simulink model "G474_Mode2_Direct_Start_Repair"  (R2024b)
settings: Solver=FixedStepDiscrete  StartTime=0.0  StopTime=q.stop_time  FixedStep=p.Ts  RelTol=1e-3
InitFcn:
  | m2_project_root=fileparts(fileparts(get_param(bdroot,'FileName')));Simulink.fileGenControl('set','CacheFolder',fullfile(m2_project_root,'work'),'CodeGenFolder',fullfile(m2_project_root,'work'),'createDir',true);m2_ws=get_param(bdroot,'ModelWorkspace');m2_q=getVariable(m2_ws,'q');if isfield(m2_q,'random_initial_angle') && m2_q.random_initial_angle,m2_q.initial_theta_e=2*pi*rand();end;m2_q.initial_state=[0;0;m2_q.initial_rpm*2*pi/60;m2_q.initial_theta_e];assignin(m2_ws,'q',m2_q);fprintf('MODE2 physical initial electrical angle: %.9f deg (random=%d)\n',m2_q.initial_theta_e*180/pi,m2_q.random_initial_angle);
model workspace (MAT data in the model file):
  fSin = [0 0.00153398001567 0.00306795700453 0.00460192607716 0.00613588513806 0.00766982883215 0.00920375529677 0.0107376594096 0.0122715383768 0.0138053894043 0.0153392059729 0.0168729871511 ... (1025 elements, 1025x1)]
  p.Rs = 0.875
  p.Ls = 0.0002
  p.Ld = 0.0002
  p.Lq = 0.0002
  p.Flux = 0.00752
  p.MOTOR_POLES = 14
  p.Ts = 5e-05
  p.Gain = 5000
  p.PLL_BW_Hz = 15
  p.Comp_BW_Hz = 5
  p.PLL_kp = 188.495559215
  p.PLL_ki = 0.444132198049
  p.Comp_Kp = 62.8318530718
  p.Comp_Ki = 0.0493480220054
  p.Comp_Mode = 0
  p.SMO_Kslide = 10
  p.SMO_Boundary = 0.002
  p.V_deadtime = 0.3
  p.current_deadband = 0.01
  p.pll_step_limit = 0.157079632679
  p.speed_decimation = 8
  p.speed_filter_old = 0.95
  p.speed_filter_new = 0.05
  q.Ts = 5e-05
  q.Rs = 0.875
  q.Ld = 0.0002
  q.Lq = 0.0002
  q.Flux = 0.00752
  q.pole_pairs = 7
  q.target_rpm = 200
  q.second_rpm = 400
  q.third_rpm = 1000
  q.switch_1 = 0.8
  q.switch_2 = 1.6
  q.Vbus = 12
  q.stop_time = 4
  q.J = 2e-05
  q.B = 1e-05
  q.load_torque = 0.005
  q.load_speed_scale_rad_s = 1
  q.random_initial_angle = 1
  q.initial_theta_e = 0.523598775598
  q.initial_rpm = 0
  q.actual_deadtime_V = 0.3
  q.observer_deadtime_V = 0.3
  q.speed_iq_sign = 1
  q.deadtime_feedforward_V = 0.3
  q.feedforward_start_s = 0.5
  q.feedforward_ramp_s = 0.5
  q.speed_kp = 0.01
  q.speed_ki = 0.0001
  q.current_kp = 0.01
  q.current_ki = 1e-05
  q.iq_limit = 12
  q.reference_filter_hz = 2
  q.reference_start_delay_s = 0.15
  q.ramp_step = 0.05
  q.current_channel_sign = 1
  q.initial_state = [0; 0; 0; 0.523598775598]
  s0.psi_s = [0; 0]
  s0.theta = 0
(part 1 of 2)
settings Model: Creator=QXZ-030079  LastModifiedBy=QXZ-030079
settings DataIOCC: SignalLogging=off

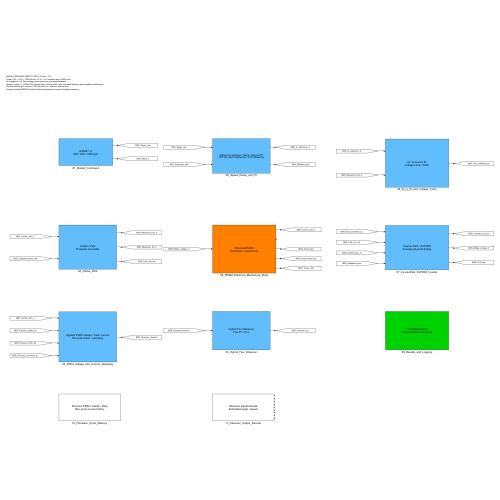
[thumbnail: Simulink's stored preview of the top-level diagram]
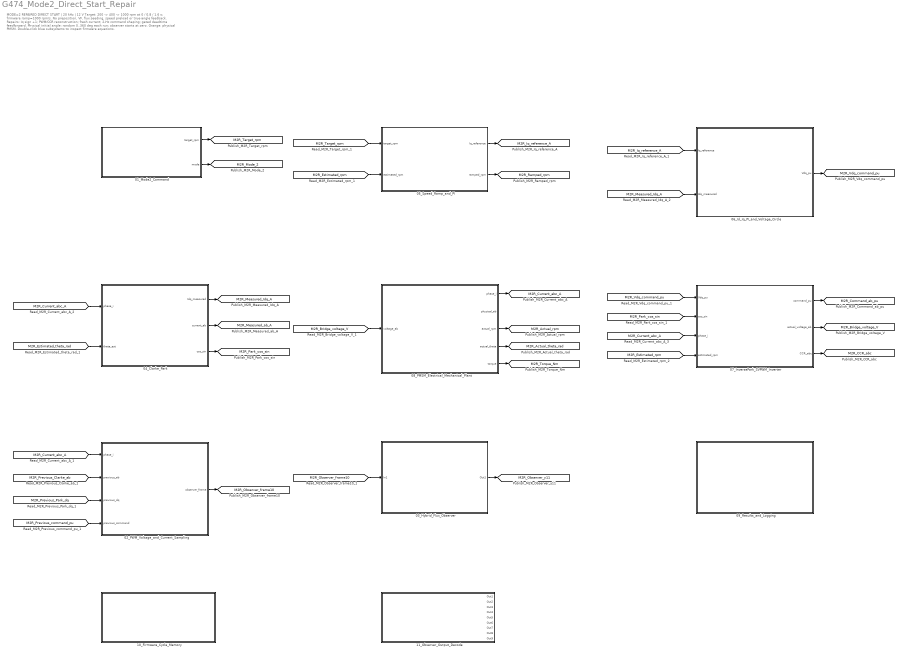
== system G474_Mode2_Direct_Start_Repair ==
  note: MODE=2 REPAIRED DIRECT START | 20 kHz | 12 V
      | Target: 200 -> 400 -> 1000 rpm at 0 / 0.8 / 1.6 s; firmware ramp=1000 rpm/s.
      | No preposition, VF, flux seeding, speed preload or true-angle feedback.
      | Repairs: Iq sign +1; PWM/CCR reconstruction; fresh current; 2-Hz command shaping; gated deadtime feedforward.
      | Physical initial angle: random 0..360 deg each run; observer starts at zero.
      | Orange: physical PMSM. Double-click blue subsystems to inspect firmware equations.
  01_Mode2_Command : Subsystem
      mask Display: disp('MODE = 2\n200 / 400 / 1000 rpm');
  02_PWM_Voltage_and_Current_Sampling : Subsystem
      mask Display: disp('Applied PWM voltage / fresh current\nReconstruction / sampling');
  03_Hybrid_Flux_Observer : Subsystem
      settings: OpenFcn=open_system(gcb,'force')
      mask Display: disp('Hybrid Flux Observer\nFlux PI + PLL');
  04_Clarke_Park : Subsystem
      mask Display: disp('Clarke / Park\nFirmware sine table');
  05_Speed_Ramp_and_PI : Subsystem
      mask Display: disp('Observer warmup / ramp / source PI\n150 ms zero reference / 2 Hz shaping');
  06_Id_Iq_PI_and_Voltage_Circle : Subsystem
      mask Display: disp('Id / Iq source PI\nVoltage circle / OutF');
  07_InversePark_SVPWM_Inverter : Subsystem
      mask Display: disp('Inverse Park / SVPWM\nAverage physical bridge');
  08_PMSM_Electrical_Mechanical_Plant : Subsystem
      mask Display: disp('Physical PMSM\nElectrical + mechanical');
  09_Results_and_Logging : Subsystem
      mask Display: disp('11 labelled scopes\nActual / estimated results');
  10_Firmware_Cycle_Memory : Subsystem
      mask Display: disp('Previous PWM / Clarke / Park\nOne-cycle source history');
  11_Observer_Output_Decode : Subsystem
      mask Display: disp('Observer signal decode\nEstimated angle / speed');
  tag scope: M2R_Actual_rpm=global, M2R_Actual_theta_rad=global, M2R_Bridge_voltage_V=global, M2R_CCR_abc=global, M2R_Command_ab_pu=global, M2R_Current_abc_A=global, M2R_Iq_reference_A=global, M2R_Measured_Idq_A=global, M2R_Measured_ab_A=global, M2R_Mode_2=global, M2R_Observer_frame10=global, M2R_Observer_y11=global, M2R_Park_cos_sin=global, M2R_Ramped_rpm=global, M2R_Target_rpm=global, M2R_Torque_Nm=global, M2R_Vdq_command_pu=global
  wires:
  01_Mode2_Command/2(mode) -> [M2R_Mode_2]
  07_InversePark_SVPWM_Inverter/3(CCR_abc) -> [M2R_CCR_abc]
  05_Speed_Ramp_and_PI/2(ramped_rpm) -> [M2R_Ramped_rpm]
  08_PMSM_Electrical_Mechanical_Plant/5(torque) -> [M2R_Torque_Nm]
  08_PMSM_Electrical_Mechanical_Plant/4(actual_theta) -> [M2R_Actual_theta_rad]
  08_PMSM_Electrical_Mechanical_Plant/3(actual_rpm) -> [M2R_Actual_rpm]
  07_InversePark_SVPWM_Inverter/2(actual_voltage_ab) -> [M2R_Bridge_voltage_V]
  [M2R_Bridge_voltage_V] -> 08_PMSM_Electrical_Mechanical_Plant/1(voltage_ab)
  04_Clarke_Park/3(cos_sin) -> [M2R_Park_cos_sin]
  [M2R_Park_cos_sin] -> 07_InversePark_SVPWM_Inverter/2(cos_sin)
  06_Id_Iq_PI_and_Voltage_Circle/1(Vdq_pu) -> [M2R_Vdq_command_pu]
  [M2R_Vdq_command_pu] -> 07_InversePark_SVPWM_Inverter/1(Vdq_pu)
  05_Speed_Ramp_and_PI/1(Iq_reference) -> [M2R_Iq_reference_A]
  [M2R_Iq_reference_A] -> 06_Id_Iq_PI_and_Voltage_Circle/1(Iq_reference)
  [M2R_Estimated_rpm] -> 05_Speed_Ramp_and_PI/2(estimated_rpm)
  [M2R_Estimated_rpm] -> 07_InversePark_SVPWM_Inverter/4(estimated_rpm)
  01_Mode2_Command/1(target_rpm) -> [M2R_Target_rpm]
  [M2R_Target_rpm] -> 05_Speed_Ramp_and_PI/1(target_rpm)
  [M2R_Estimated_theta_rad] -> 04_Clarke_Park/2(theta_est)
  03_Hybrid_Flux_Observer/1(Out1) -> [M2R_Observer_y11]
  02_PWM_Voltage_and_Current_Sampling/1(observer_frame) -> [M2R_Observer_frame10]
  [M2R_Observer_frame10] -> 03_Hybrid_Flux_Observer/1(In1)
  [M2R_Previous_command_pu] -> 02_PWM_Voltage_and_Current_Sampling/4(previous_command)
  [M2R_Previous_Park_dq] -> 02_PWM_Voltage_and_Current_Sampling/3(previous_dq)
  [M2R_Previous_Clarke_ab] -> 02_PWM_Voltage_and_Current_Sampling/2(previous_ab)
  08_PMSM_Electrical_Mechanical_Plant/1(phase_i) -> [M2R_Current_abc_A]
  [M2R_Current_abc_A] -> 02_PWM_Voltage_and_Current_Sampling/1(phase_i)
  [M2R_Current_abc_A] -> 04_Clarke_Park/1(phase_i)
  [M2R_Current_abc_A] -> 07_InversePark_SVPWM_Inverter/3(phase_i)
  04_Clarke_Park/1(Idq_measured) -> [M2R_Measured_Idq_A]
  [M2R_Measured_Idq_A] -> 06_Id_Iq_PI_and_Voltage_Circle/2(Idq_measured)
  04_Clarke_Park/2(current_ab) -> [M2R_Measured_ab_A]
  07_InversePark_SVPWM_Inverter/1(command_pu) -> [M2R_Command_ab_pu]

== system G474_Mode2_Direct_Start_Repair/01_Mode2_Command ==
  Initial_200rpm : Constant  Value=q.target_rpm
  MODE_SENSORLESS_2 : Constant  Value=2
  Speed_schedule : Sum  Inputs=+++
  Switch_to_1000rpm : Step  Time=q.switch_2  After=q.third_rpm-q.second_rpm  SampleTime=p.Ts
  Switch_to_400rpm : Step  Time=q.switch_1  After=q.second_rpm-q.target_rpm  SampleTime=p.Ts
  target_rpm : Outport
  mode : Outport  Port=2
  wires:
  MODE_SENSORLESS_2/1 -> mode/1
  Speed_schedule/1 -> target_rpm/1
  Initial_200rpm/1 -> Speed_schedule/1
  Switch_to_400rpm/1 -> Speed_schedule/2
  Switch_to_1000rpm/1 -> Speed_schedule/3

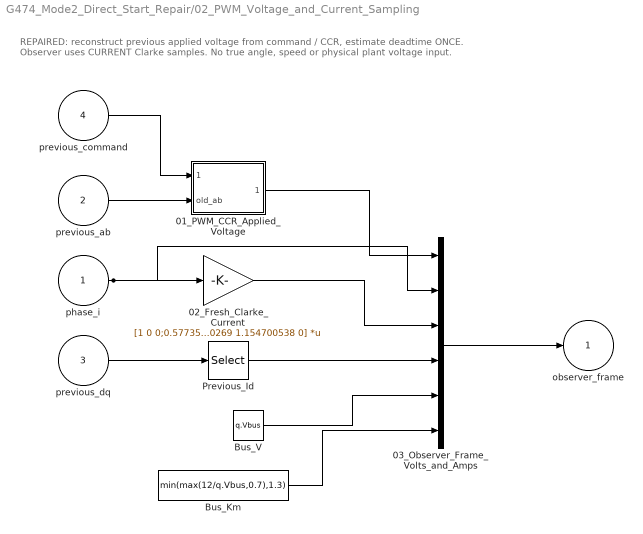
== system G474_Mode2_Direct_Start_Repair/02_PWM_Voltage_and_Current_Sampling ==
  note: REPAIRED: reconstruct previous applied voltage from command / CCR, estimate deadtime ONCE.
      | Observer uses CURRENT Clarke samples. No true angle, speed or physical plant voltage input.
  phase_i : Inport
  previous_ab : Inport  Port=2
  previous_dq : Inport  Port=3
  previous_command : Inport  Port=4
  01_PWM_CCR_Applied_Voltage : MATLAB Function  TreatAsAtomicUnit=on
  02_Fresh_Clarke_Current : Gain  Gain=[1 0 0;0.577350269 1.154700538 0]  Multiplication=Matrix(K*u)
  03_Observer_Frame_Volts_and_Amps : Mux  Inputs=6
  Bus_Km : Constant  Value=min(max(12/q.Vbus,0.7),1.3)
  Bus_V : Constant  Value=q.Vbus
  Previous_Id : Selector  InputPortWidth=2  IndexOptions=Index vector (dialog)  Indices=1  OutputSizes=1
  observer_frame : Outport
  wires:
  01_PWM_CCR_Applied_Voltage/1(voltage) -> 03_Observer_Frame_Volts_and_Amps/1
  previous_command/1 -> 01_PWM_CCR_Applied_Voltage/1(old_command)
  Previous_Id/1 -> 03_Observer_Frame_Volts_and_Amps/4
  Bus_V/1 -> 03_Observer_Frame_Volts_and_Amps/5
  previous_ab/1 -> 01_PWM_CCR_Applied_Voltage/2(old_ab)
  phase_i/1 -> 03_Observer_Frame_Volts_and_Amps/2, 02_Fresh_Clarke_Current/1
  previous_dq/1 -> Previous_Id/1
  02_Fresh_Clarke_Current/1 -> 03_Observer_Frame_Volts_and_Amps/3
  Bus_Km/1 -> 03_Observer_Frame_Volts_and_Amps/6
  03_Observer_Frame_Volts_and_Amps/1 -> observer_frame/1

== system G474_Mode2_Direct_Start_Repair/03_Hybrid_Flux_Observer ==
  In1 : Inport
  01_Voltage_Compensation : Subsystem
      settings: OpenFcn=open_system(gcb,'force')
      mask Display: port_label('input',1,'command_pu');port_label('input',2,'phase_current');port_label('input',3,'Vbus');port_label('input',4,'Km');port_label('output',1,'voltage_V');
  02_Active_Flux_Models : Subsystem
      settings: OpenFcn=open_system(gcb,'force')
      mask Display: port_label('input',1,'theta_previous');port_label('input',2,'current_ab');port_label('input',3,'psi_s_previous');port_label('input',4,'Id');port_label('output',1,'psi_I');port_label('output',2,'psi_V');
  03_Flux_Feedback : Subsystem
      settings: OpenFcn=open_system(gcb,'force')
      mask Display: port_label('input',1,'psi_I');port_label('input',2,'psi_V');port_label('output',1,'Ucomp');
  04_Stator_Integrator : Subsystem
      settings: OpenFcn=open_system(gcb,'force')
      mask Display: port_label('input',1,'voltage_V');port_label('input',2,'current_ab');port_label('input',3,'Ucomp');port_label('output',1,'psi_s_new');port_label('output',2,'psi_s_previous');
  05_PLL_and_Angle : Subsystem
      settings: OpenFcn=open_system(gcb,'force')
      mask Display: port_label('input',1,'psi_V');port_label('output',1,'theta_previous');port_label('output',2,'step_rad');port_label('output',3,'theta_new');port_label('output',4,'PLL_error');
  06_Speed_Filter : Subsystem
      settings: OpenFcn=open_system(gcb,'force')
      mask Display: port_label('input',1,'step_rad');port_label('output',1,'electrical_Hz');port_label('output',2,'firmware_RPM');
  Input split : Demux  Outputs=[2 3 2 1 1 1]
  Results : Mux  Inputs=8
  Out1 : Outport
  wires:
  03_Flux_Feedback/1(Ucomp) -> 04_Stator_Integrator/3(Ucomp)
  02_Active_Flux_Models/2(psi_V) -> 05_PLL_and_Angle/1(psi_V), Results/4, 03_Flux_Feedback/2(psi_V)
  06_Speed_Filter/2(firmware_RPM) -> Results/3
  06_Speed_Filter/1(electrical_Hz) -> Results/2
  Results/1 -> Out1/1
  04_Stator_Integrator/2(psi_s_previous) -> 02_Active_Flux_Models/3(psi_s_previous)
  04_Stator_Integrator/1(psi_s_new) -> Results/5
  05_PLL_and_Angle/4(PLL_error) -> Results/6
  05_PLL_and_Angle/3(theta_new) -> Results/1
  05_PLL_and_Angle/2(step_rad) -> 06_Speed_Filter/1(step_rad), Results/7
  02_Active_Flux_Models/1(psi_I) -> 03_Flux_Feedback/1(psi_I)
  Input split/3 -> 02_Active_Flux_Models/2(current_ab), 04_Stator_Integrator/2(current_ab)
  Input split/4 -> 02_Active_Flux_Models/4(Id)
  In1/1 -> Input split/1
  05_PLL_and_Angle/1(theta_previous) -> 02_Active_Flux_Models/1(theta_previous)
  Input split/1 -> 01_Voltage_Compensation/1(input1)
  Input split/2 -> 01_Voltage_Compensation/2(input2)
  Input split/5 -> 01_Voltage_Compensation/3(input3)
  Input split/6 -> 01_Voltage_Compensation/4(input4)
  01_Voltage_Compensation/1(Applied_voltage_V) -> 04_Stator_Integrator/1(voltage_V), Results/8

== system G474_Mode2_Direct_Start_Repair/04_Clarke_Park ==
  phase_i : Inport
  theta_est : Inport  Port=2
  Source_lookup_and_transform : MATLAB Function  TreatAsAtomicUnit=on
  Idq_measured : Outport
  current_ab : Outport  Port=2
  cos_sin : Outport  Port=3
  wires:
  phase_i/1 -> Source_lookup_and_transform/1(iabc)
  Source_lookup_and_transform/3(cs) -> cos_sin/1
  theta_est/1 -> Source_lookup_and_transform/2(theta)
  Source_lookup_and_transform/1(dq) -> Idq_measured/1
  Source_lookup_and_transform/2(iab) -> current_ab/1

== system G474_Mode2_Direct_Start_Repair/05_Speed_Ramp_and_PI ==
  note: MODE=2 throughout: zero reference for 150 ms while observer states naturally converge.
      | No alignment current, VF, true angle or flux preset. Then 2-pole 2-Hz shaping and source slew limiter.
      | PI gains/anti-windup equations, PLL and speed filter remain unchanged.
  target_rpm : Inport
  estimated_rpm : Inport  Port=2
  01_Observer_Warmup_and_Command_Shaping : Subsystem
      mask Display: disp('Zero-reference warmup 150 ms\nThen two 2-Hz reference filters');
  02_Speed_Slew_Limiter : Subsystem
      mask Display: disp('Speed slew limiter\n1000 rpm per second');
  03_Speed_PI_Output_and_Polarity : Subsystem
      mask Display: disp('Source speed PI / OutF\nIq limit 12 A / polarity +1');
  Iq_reference : Outport
  ramped_rpm : Outport  Port=2
  wires:
  03_Speed_PI_Output_and_Polarity/1(Out1) -> Iq_reference/1
  target_rpm/1 -> 01_Observer_Warmup_and_Command_Shaping/1(In1)
  01_Observer_Warmup_and_Command_Shaping/1(Out1) -> 02_Speed_Slew_Limiter/2(In2)
  estimated_rpm/1 -> 03_Speed_PI_Output_and_Polarity/1(Fbk)
  02_Speed_Slew_Limiter/1(Out1) -> 02_Speed_Slew_Limiter/1(In1), ramped_rpm/1, 03_Speed_PI_Output_and_Polarity/2(Ref)

== system G474_Mode2_Direct_Start_Repair/06_Id_Iq_PI_and_Voltage_Circle ==
  Iq_reference : Inport
  Idq_measured : Inport  Port=2
  01_Id_PI_and_Filter : Subsystem
      mask Display: disp('d-axis source PI\nId = 0 A / OutF');
  02_Voltage_Circle : Subsystem
      mask Display: disp('Voltage circle\nsqrt(limit^2 - Vd^2)');
  03_Iq_PI_and_Filter : Subsystem
      mask Display: disp('q-axis source PI\nDynamic voltage limits / OutF');
  Split_Id_Iq : Demux  Outputs=2
  Vd_Vq : Mux  Inputs=2
  Vdq_pu : Outport
  wires:
  Split_Id_Iq/1 -> 01_Id_PI_and_Filter/2(Fbk)
  Idq_measured/1 -> Split_Id_Iq/1
  02_Voltage_Circle/1(Out1) -> 03_Iq_PI_and_Filter/2(Umax)
  Split_Id_Iq/2 -> 03_Iq_PI_and_Filter/3(Fbk)
  01_Id_PI_and_Filter/1(Out1) -> 01_Id_PI_and_Filter/1(In1), Vd_Vq/1, 02_Voltage_Circle/1(In1)
  Iq_reference/1 -> 03_Iq_PI_and_Filter/1(Ref)
  02_Voltage_Circle/2(Out2) -> 03_Iq_PI_and_Filter/4(Umin)
  03_Iq_PI_and_Filter/1(Out1) -> Vd_Vq/2
  Vd_Vq/1 -> Vdq_pu/1

== system G474_Mode2_Direct_Start_Repair/07_InversePark_SVPWM_Inverter ==
  note: Inverter deadtime feedforward: measured current polarity -> voltage-loss estimate -> PWM command.
      | Source SVPWM sector / CCR truncation / 0..3999 clamp retained.
      | Physical voltage is independently reconstructed from duty ratios and physical deadtime.
  Vdq_pu : Inport
  cos_sin : Inport  Port=2
  phase_i : Inport  Port=3
  estimated_rpm : Inport  Port=4
  Deadtime_Voltage_Feedforward : MATLAB Function  TreatAsAtomicUnit=on
  Inverse_Park : MATLAB Function  TreatAsAtomicUnit=on
  Mode2_elapsed_time : DigitalClock  SampleTime=p.Ts
  Source_SVPWM_and_average_bridge : MATLAB Function  TreatAsAtomicUnit=on
  command_pu : Outport
  actual_voltage_ab : Outport  Port=2
  CCR_abc : Outport  Port=3
  wires:
  Vdq_pu/1 -> Inverse_Park/1(vdq)
  estimated_rpm/1 -> Deadtime_Voltage_Feedforward/3(estimated_rpm)
  cos_sin/1 -> Inverse_Park/2(cs)
  Mode2_elapsed_time/1 -> Deadtime_Voltage_Feedforward/4(time)
  Inverse_Park/1(command) -> Deadtime_Voltage_Feedforward/1(desired_command)
  Deadtime_Voltage_Feedforward/1(applied_command) -> Source_SVPWM_and_average_bridge/1(command), command_pu/1
  phase_i/1 -> Source_SVPWM_and_average_bridge/2(iabc), Deadtime_Voltage_Feedforward/2(phase_i)
  Source_SVPWM_and_average_bridge/1(voltage) -> actual_voltage_ab/1
  Source_SVPWM_and_average_bridge/2(ccr) -> CCR_abc/1

== system G474_Mode2_Direct_Start_Repair/08_PMSM_Electrical_Mechanical_Plant ==
  note: True angle/speed are used only by the physical plant and result plots.
      | J=2e-5 kg*m^2, B=1e-5 N*m*s/rad: assumed.
      | Default load=0.005*tanh(wm/1) Nm, opposing motion; zero scale selects fixed external torque.
      | Initial speed/current=0; initial electrical angle=30 deg; observer state=0.
  voltage_ab : Inport
  Electrical_and_mechanical_RK4 : MATLAB Function  TreatAsAtomicUnit=on
  Physical_measurements : MATLAB Function  TreatAsAtomicUnit=on
  Physical_state_id_iq_wm_theta : UnitDelay  InitialCondition=q.initial_state  SampleTime=p.Ts  HasFrameUpgradeWarning=on
  phase_i : Outport
  physical_ab : Outport  Port=2
  actual_rpm : Outport  Port=3
  actual_theta : Outport  Port=4
  torque : Outport  Port=5
  wires:
  Physical_measurements/2(iab) -> physical_ab/1
  voltage_ab/1 -> Electrical_and_mechanical_RK4/2(v)
  Electrical_and_mechanical_RK4/1(xn) -> Physical_state_id_iq_wm_theta/1
  Physical_state_id_iq_wm_theta/1 -> Electrical_and_mechanical_RK4/1(x), Physical_measurements/1(x)
  Physical_measurements/1(iabc) -> phase_i/1
  Physical_measurements/3(rpm) -> actual_rpm/1
  Physical_measurements/4(theta) -> actual_theta/1
  Physical_measurements/5(torque) -> torque/1

== system G474_Mode2_Direct_Start_Repair/09_Results_and_Logging ==
  09_Results_11_Scopes : Subsystem
  Logging_taps : Subsystem
  tag scope: M2R_Full_log34=global
  wires:
  [M2R_Full_log34] -> 09_Results_11_Scopes/1(signals34)
  Logging_taps/1(Out1) -> [M2R_Full_log34]

== system G474_Mode2_Direct_Start_Repair/10_Firmware_Cycle_Memory ==
  Previous_Clarke_ab : UnitDelay  InitialCondition=[0;0]  SampleTime=p.Ts  HasFrameUpgradeWarning=on
  Previous_Park_dq : UnitDelay  InitialCondition=[0;0]  SampleTime=p.Ts  HasFrameUpgradeWarning=on
  Previous_command_pu : UnitDelay  InitialCondition=[0;0]  SampleTime=p.Ts  HasFrameUpgradeWarning=on
  tag scope: M2R_Previous_Clarke_ab=global, M2R_Previous_Park_dq=global, M2R_Previous_command_pu=global
  wires:
  [M2R_Measured_ab_A] -> Previous_Clarke_ab/1
  [M2R_Command_ab_pu] -> Previous_command_pu/1
  [M2R_Measured_Idq_A] -> Previous_Park_dq/1
  Previous_Clarke_ab/1 -> [M2R_Previous_Clarke_ab]
  Previous_command_pu/1 -> [M2R_Previous_command_pu]
  Previous_Park_dq/1 -> [M2R_Previous_Park_dq]

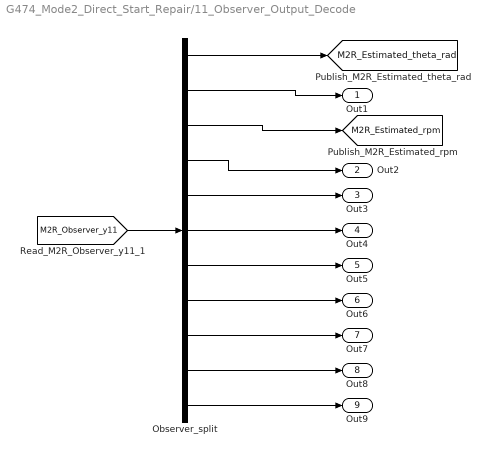
== system G474_Mode2_Direct_Start_Repair/11_Observer_Output_Decode ==
  Observer_split : Demux  Outputs=11
  Out1 : Outport
  Out2 : Outport  Port=2
  Out3 : Outport  Port=3
  Out4 : Outport  Port=4
  Out5 : Outport  Port=5
  Out6 : Outport  Port=6
  Out7 : Outport  Port=7
  Out8 : Outport  Port=8
  Out9 : Outport  Port=9
  tag scope: M2R_Estimated_rpm=global, M2R_Estimated_theta_rad=global
  wires:
  [M2R_Observer_y11] -> Observer_split/1
  Observer_split/1 -> [M2R_Estimated_theta_rad]
  Observer_split/2 -> Out1/1
  Observer_split/3 -> [M2R_Estimated_rpm]
  Observer_split/4 -> Out2/1
  Observer_split/5 -> Out3/1
  Observer_split/6 -> Out4/1
  Observer_split/7 -> Out5/1
  Observer_split/8 -> Out6/1
  Observer_split/9 -> Out7/1
  Observer_split/10 -> Out8/1
  Observer_split/11 -> Out9/1

== system G474_Mode2_Direct_Start_Repair/03_Hybrid_Flux_Observer/01_Voltage_Compensation ==
  note: Applied VOLTS reconstructed upstream from PWM and measured current.
      | No second bus scaling or deadtime correction. PI equations and gains remain source values.
  input1 : Inport
  input2 : Inport  Port=2
  input3 : Inport  Port=3
  input4 : Inport  Port=4
  Unused_legacy_port2 : Terminator
  Unused_legacy_port3 : Terminator
  Unused_legacy_port4 : Terminator
  Applied_voltage_V : Outport
  wires:
  input2/1 -> Unused_legacy_port2/1
  input4/1 -> Unused_legacy_port4/1
  input1/1 -> Applied_voltage_V/1
  input3/1 -> Unused_legacy_port3/1

== system G474_Mode2_Direct_Start_Repair/03_Hybrid_Flux_Observer/02_Active_Flux_Models ==
  theta_previous : Inport
  current_ab : Inport  Port=2
  psi_s_previous : Inport  Port=3
  Id : Inport  Port=4
  Current model : Subsystem
      settings: OpenFcn=open_system(gcb,'force')
      mask Display: port_label('input',1,'theta_previous');port_label('input',2,'Id');port_label('output',1,'psi_I');
  Voltage model extraction : Subsystem
      settings: OpenFcn=open_system(gcb,'force')
      mask Display: port_label('input',1,'psi_s_previous');port_label('input',2,'current_ab');port_label('output',1,'psi_V');
  psi_I : Outport
  psi_V : Outport  Port=2
  wires:
  psi_s_previous/1 -> Voltage model extraction/1(psi_s_previous)
  Current model/1(psi_I) -> psi_I/1
  current_ab/1 -> Voltage model extraction/2(current_ab)
  Id/1 -> Current model/2(Id)
  Voltage model extraction/1(psi_V) -> psi_V/1
  theta_previous/1 -> Current model/1(theta_previous)

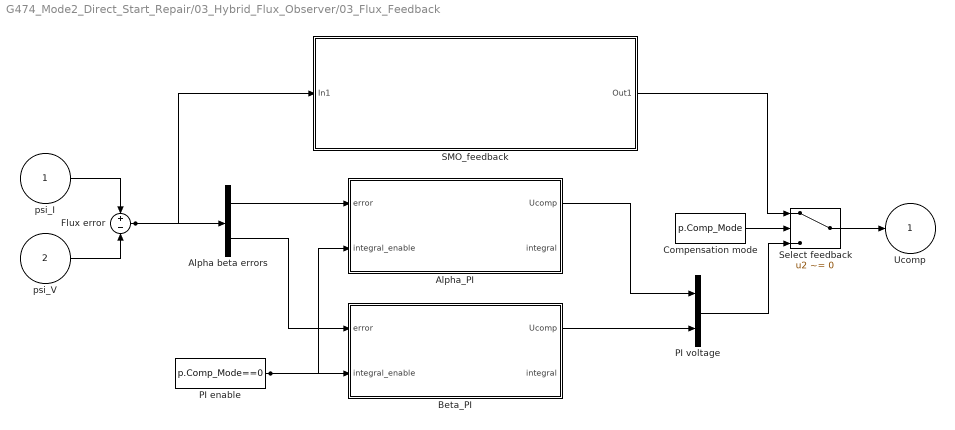
== system G474_Mode2_Direct_Start_Repair/03_Hybrid_Flux_Observer/03_Flux_Feedback ==
  psi_I : Inport
  psi_V : Inport  Port=2
  Alpha beta errors : Demux  Outputs=2
  Alpha_PI : Subsystem  mask{Kp=p.Comp_Kp, Ki=p.Comp_Ki, Ts=p.Ts}
      mask prompts: Kp "Kp (source coefficient)"; Ki "Ki (per call, already discrete)"; Ts "Execution period (s)"
      settings: OpenFcn=open_system(gcb,'force')
      mask Display: port_label('input',1,'error');port_label('input',2,'integral_enable');port_label('output',1,'Ucomp');port_label('output',2,'integral');
  Beta_PI : Subsystem  mask{Kp=p.Comp_Kp, Ki=p.Comp_Ki, Ts=p.Ts}
      mask prompts: Kp "Kp (source coefficient)"; Ki "Ki (per call, already discrete)"; Ts "Execution period (s)"
      settings: OpenFcn=open_system(gcb,'force')
      mask Display: port_label('input',1,'error');port_label('input',2,'integral_enable');port_label('output',1,'Ucomp');port_label('output',2,'integral');
  Compensation mode : Constant  Value=p.Comp_Mode
  Flux error : Sum  Inputs=+-
  PI enable : Constant  Value=p.Comp_Mode==0
  PI voltage : Mux  Inputs=2
  SMO_feedback : Subsystem
      settings: OpenFcn=open_system(gcb,'force')
      mask Display: port_label('input',1,'In1');port_label('output',1,'Out1');
  Select feedback : Switch  Criteria=u2 ~= 0  SaturateOnIntegerOverflow=off  InputSameDT=off
  Ucomp : Outport
  wires:
  Select feedback/1 -> Ucomp/1
  Compensation mode/1 -> Select feedback/2
  Beta_PI/1(Ucomp) -> PI voltage/2
  Alpha_PI/1(Ucomp) -> PI voltage/1
  SMO_feedback/1(Out1) -> Select feedback/1
  PI enable/1 -> Beta_PI/2(integral_enable), Alpha_PI/2(integral_enable)
  Alpha beta errors/2 -> Beta_PI/1(error)
  psi_V/1 -> Flux error/2
  Flux error/1 -> Alpha beta errors/1, SMO_feedback/1(In1)
  psi_I/1 -> Flux error/1
  PI voltage/1 -> Select feedback/3
  Alpha beta errors/1 -> Alpha_PI/1(error)

== system G474_Mode2_Direct_Start_Repair/03_Hybrid_Flux_Observer/04_Stator_Integrator ==
  voltage_V : Inport
  current_ab : Inport  Port=2
  Ucomp : Inport  Port=3
  Euler Ts : Gain  Gain=p.Ts
  Flux derivative : Sum  Inputs=+-+
  Resistive voltage : Gain  Gain=p.Rs
  Stator memory : UnitDelay  InitialCondition=s0.psi_s  SampleTime=p.Ts  HasFrameUpgradeWarning=on
  Updated flux : Sum
  psi_s_new : Outport
  psi_s_previous : Outport  Port=2
  wires:
  Euler Ts/1 -> Updated flux/2
  Updated flux/1 -> Stator memory/1, psi_s_new/1
  Flux derivative/1 -> Euler Ts/1
  Resistive voltage/1 -> Flux derivative/2
  Stator memory/1 -> psi_s_previous/1, Updated flux/1
  voltage_V/1 -> Flux derivative/1
  Ucomp/1 -> Flux derivative/3
  current_ab/1 -> Resistive voltage/1

== system G474_Mode2_Direct_Start_Repair/03_Hybrid_Flux_Observer/05_PLL_and_Angle ==
  psi_V : Inport
  PLL : Subsystem
      settings: OpenFcn=open_system(gcb,'force')
      mask Display: port_label('input',1,'psi_V');port_label('input',2,'theta_previous');port_label('output',1,'theta_new');port_label('output',2,'step_rad');port_label('output',3,'PLL_error');
  Previous PLL angle : UnitDelay  InitialCondition=s0.theta  SampleTime=p.Ts  HasFrameUpgradeWarning=on
  theta_previous : Outport
  step_rad : Outport  Port=2
  theta_new : Outport  Port=3
  PLL_error : Outport  Port=4
  wires:
  PLL/2(step_rad) -> step_rad/1
  psi_V/1 -> PLL/1(psi_V)
  PLL/1(theta_new) -> theta_new/1, Previous PLL angle/1
  Previous PLL angle/1 -> theta_previous/1, PLL/2(theta_previous)
  PLL/3(PLL_error) -> PLL_error/1

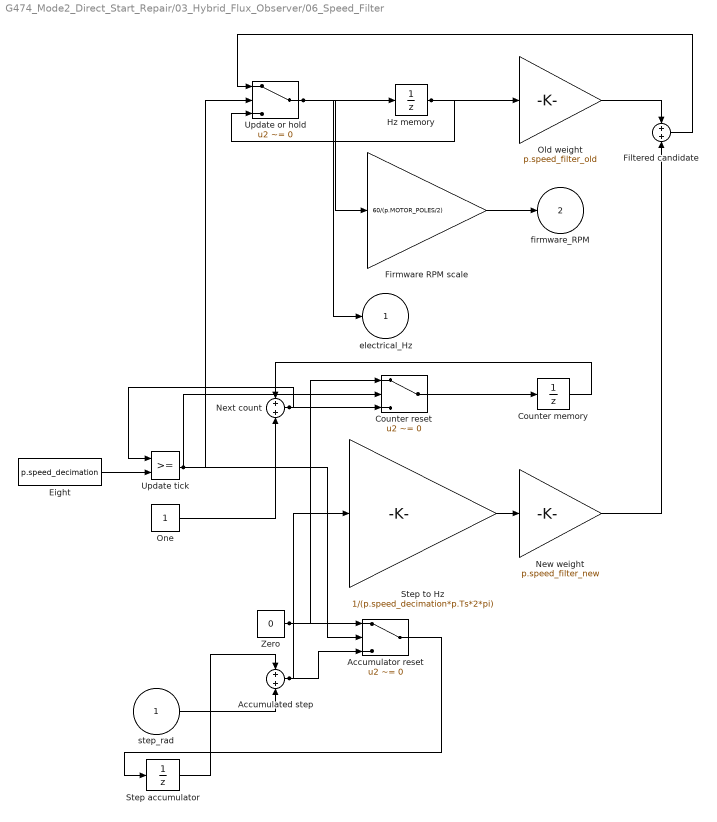
== system G474_Mode2_Direct_Start_Repair/03_Hybrid_Flux_Observer/06_Speed_Filter ==
  step_rad : Inport
  Accumulated step : Sum
  Accumulator reset : Switch  Criteria=u2 ~= 0  SaturateOnIntegerOverflow=off  InputSameDT=off
  Counter memory : UnitDelay  SampleTime=p.Ts  HasFrameUpgradeWarning=on
  Counter reset : Switch  Criteria=u2 ~= 0  SaturateOnIntegerOverflow=off  InputSameDT=off
  Eight : Constant  Value=p.speed_decimation
  Filtered candidate : Sum
  Firmware RPM scale : Gain  Gain=60/(p.MOTOR_POLES/2)
  Hz memory : UnitDelay  SampleTime=p.Ts  HasFrameUpgradeWarning=on
  New weight : Gain  Gain=p.speed_filter_new
  Next count : Sum
  Old weight : Gain  Gain=p.speed_filter_old
  One : Constant
  Step accumulator : UnitDelay  SampleTime=p.Ts  HasFrameUpgradeWarning=on
  Step to Hz : Gain  Gain=1/(p.speed_decimation*p.Ts*2*pi)
  Update or hold : Switch  Criteria=u2 ~= 0  SaturateOnIntegerOverflow=off  InputSameDT=off
  Update tick : RelationalOperator  OutDataTypeStr=boolean  RndMeth=Simplest  InputSameDT=off
  Zero : Constant  Value=0
  electrical_Hz : Outport
  firmware_RPM : Outport  Port=2
  wires:
  Filtered candidate/1 -> Update or hold/1
  New weight/1 -> Filtered candidate/2
  Counter memory/1 -> Next count/1
  Old weight/1 -> Filtered candidate/1
  Counter reset/1 -> Counter memory/1
  Hz memory/1 -> Old weight/1, Update or hold/3
  Accumulated step/1 -> Step to Hz/1, Accumulator reset/3
  Update or hold/1 -> Firmware RPM scale/1, electrical_Hz/1, Hz memory/1
  Step to Hz/1 -> New weight/1
  Step accumulator/1 -> Accumulated step/1
  step_rad/1 -> Accumulated step/2
  Firmware RPM scale/1 -> firmware_RPM/1
  Update tick/1 -> Update or hold/2, Accumulator reset/2, Counter reset/2
  Next count/1 -> Update tick/1, Counter reset/3
  Eight/1 -> Update tick/2
  One/1 -> Next count/2
  Zero/1 -> Accumulator reset/1, Counter reset/1
  Accumulator reset/1 -> Step accumulator/1

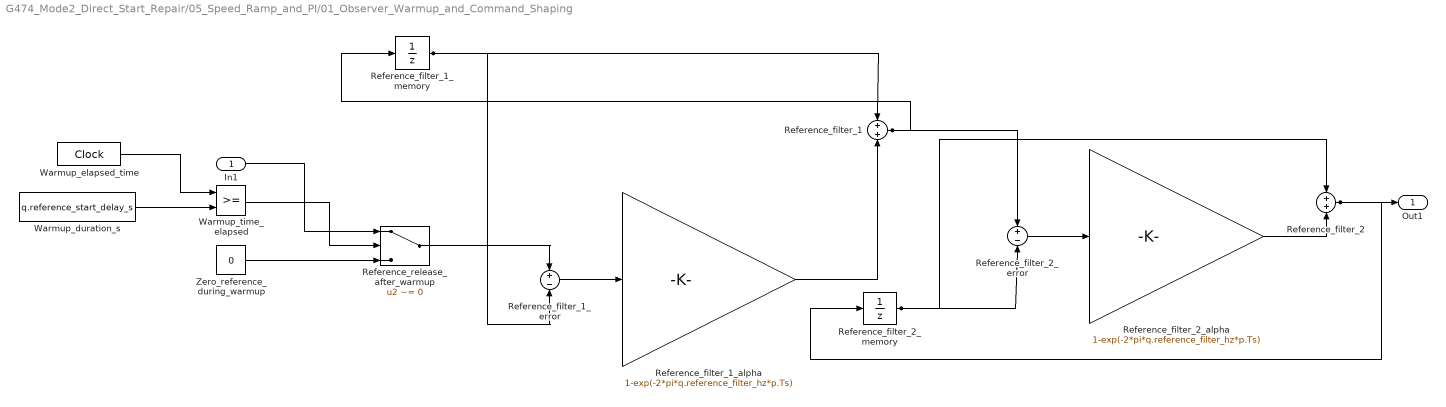
== system G474_Mode2_Direct_Start_Repair/05_Speed_Ramp_and_PI/01_Observer_Warmup_and_Command_Shaping ==
  In1 : Inport
  Reference_filter_1 : Sum
  Reference_filter_1_alpha : Gain  Gain=1-exp(-2*pi*q.reference_filter_hz*p.Ts)
  Reference_filter_1_error : Sum  Inputs=+-
  Reference_filter_1_memory : UnitDelay  SampleTime=p.Ts  HasFrameUpgradeWarning=on
  Reference_filter_2 : Sum
  Reference_filter_2_alpha : Gain  Gain=1-exp(-2*pi*q.reference_filter_hz*p.Ts)
  Reference_filter_2_error : Sum  Inputs=+-
  Reference_filter_2_memory : UnitDelay  SampleTime=p.Ts  HasFrameUpgradeWarning=on
  Reference_release_after_warmup : Switch  Criteria=u2 ~= 0  SaturateOnIntegerOverflow=off  InputSameDT=off
  Warmup_duration_s : Constant  Value=q.reference_start_delay_s
  Warmup_elapsed_time : DigitalClock  SampleTime=p.Ts
  Warmup_time_elapsed : RelationalOperator  OutDataTypeStr=boolean  RndMeth=Simplest  InputSameDT=off
  Zero_reference_during_warmup : Constant  Value=0
  Out1 : Outport
  wires:
  Warmup_elapsed_time/1 -> Warmup_time_elapsed/1
  Zero_reference_during_warmup/1 -> Reference_release_after_warmup/3
  Warmup_duration_s/1 -> Warmup_time_elapsed/2
  Warmup_time_elapsed/1 -> Reference_release_after_warmup/2
  In1/1 -> Reference_release_after_warmup/1
  Reference_filter_1_memory/1 -> Reference_filter_1_error/2, Reference_filter_1/1
  Reference_release_after_warmup/1 -> Reference_filter_1_error/1
  Reference_filter_1_error/1 -> Reference_filter_1_alpha/1
  Reference_filter_1_alpha/1 -> Reference_filter_1/2
  Reference_filter_1/1 -> Reference_filter_1_memory/1, Reference_filter_2_error/1
  Reference_filter_2_memory/1 -> Reference_filter_2_error/2, Reference_filter_2/1
  Reference_filter_2_error/1 -> Reference_filter_2_alpha/1
  Reference_filter_2_alpha/1 -> Reference_filter_2/2
  Reference_filter_2/1 -> Reference_filter_2_memory/1, Out1/1

== system G474_Mode2_Direct_Start_Repair/05_Speed_Ramp_and_PI/02_Speed_Slew_Limiter ==
  In1 : Inport
  In2 : Inport  Port=2
  Previous_ramped_rpm : UnitDelay  SampleTime=p.Ts  HasFrameUpgradeWarning=on
  Ramp_error : Sum  Inputs=+-
  Ramp_update : Sum
  Source_ramp_1000rpm_per_second : Saturate  UpperLimit=q.ramp_step  LowerLimit=-q.ramp_step
  Out1 : Outport
  wires:
  Previous_ramped_rpm/1 -> Ramp_error/2, Ramp_update/1
  In1/1 -> Previous_ramped_rpm/1
  In2/1 -> Ramp_error/1
  Ramp_error/1 -> Source_ramp_1000rpm_per_second/1
  Source_ramp_1000rpm_per_second/1 -> Ramp_update/2
  Ramp_update/1 -> Out1/1

== system G474_Mode2_Direct_Start_Repair/05_Speed_Ramp_and_PI/03_Speed_PI_Output_and_Polarity ==
  Fbk : Inport
  Ref : Inport  Port=2
  Iq_Torque_Polarity_plus1 : Gain  Gain=q.speed_iq_sign
  Lower_minus12A : Constant  Value=-q.iq_limit
  Speed_OutF : Sum
  Speed_OutF_new_01 : Gain  Gain=0.1
  Speed_OutF_old_09 : Gain  Gain=0.9
  Speed_OutF_previous : UnitDelay  SampleTime=p.Ts  HasFrameUpgradeWarning=on
  Speed_PI : Subsystem  mask{Kp=q.speed_kp, Ki=q.speed_ki, Ts=p.Ts}
      mask prompts: Kp "Kp (source coefficient)"; Ki "Ki (per call, already discrete)"; Ts "Execution period (s)"
      settings: OpenFcn=open_system(gcb,'force')
      mask Display: port_label('input',1,'Ref');port_label('input',2,'Fbk');port_label('input',3,'Umax');port_label('input',4,'Umin');port_label('output',1,'Out');port_label('output',2,'ui');port_label('output',3,'v1');port_label('output',4,'up');
  Upper_12A : Constant  Value=q.iq_limit
  Out1 : Outport
  wires:
  Lower_minus12A/1 -> Speed_PI/4(Umin)
  Ref/1 -> Speed_PI/1(Ref)
  Fbk/1 -> Speed_PI/2(Fbk)
  Upper_12A/1 -> Speed_PI/3(Umax)
  Speed_PI/1(Out) -> Speed_OutF_new_01/1
  Speed_OutF_new_01/1 -> Speed_OutF/2
  Speed_OutF_previous/1 -> Speed_OutF_old_09/1
  Speed_OutF_old_09/1 -> Speed_OutF/1
  Speed_OutF/1 -> Speed_OutF_previous/1, Iq_Torque_Polarity_plus1/1
  Iq_Torque_Polarity_plus1/1 -> Out1/1

== system G474_Mode2_Direct_Start_Repair/06_Id_Iq_PI_and_Voltage_Circle/01_Id_PI_and_Filter ==
  In1 : Inport
  Fbk : Inport  Port=2
  Bus_voltage_limit : Constant  Value=min(max(q.Vbus/12,0),0.95)
  Id_OutF : Sum
  Id_OutF_new_01 : Gain  Gain=0.1
  Id_OutF_old_09 : Gain  Gain=0.9
  Id_OutF_previous : UnitDelay  SampleTime=p.Ts  HasFrameUpgradeWarning=on
  Id_PI : Subsystem  mask{Kp=q.current_kp, Ki=q.current_ki, Ts=p.Ts}
      mask prompts: Kp "Kp (source coefficient)"; Ki "Ki (per call, already discrete)"; Ts "Execution period (s)"
      settings: OpenFcn=open_system(gcb,'force')
      mask Display: port_label('input',1,'Ref');port_label('input',2,'Fbk');port_label('input',3,'Umax');port_label('input',4,'Umin');port_label('output',1,'Out');port_label('output',2,'ui');port_label('output',3,'v1');port_label('output',4,'up');
  Id_reference_zero : Constant  Value=0
  Negative_bus_limit : Constant  Value=-min(max(q.Vbus/12,0),0.95)
  Out1 : Outport
  wires:
  In1/1 -> Id_OutF_previous/1
  Id_reference_zero/1 -> Id_PI/1(Ref)
  Id_OutF_previous/1 -> Id_OutF_old_09/1
  Fbk/1 -> Id_PI/2(Fbk)
  Bus_voltage_limit/1 -> Id_PI/3(Umax)
  Negative_bus_limit/1 -> Id_PI/4(Umin)
  Id_OutF_new_01/1 -> Id_OutF/2
  Id_PI/1(Out) -> Id_OutF_new_01/1
  Id_OutF_old_09/1 -> Id_OutF/1
  Id_OutF/1 -> Out1/1

== system G474_Mode2_Direct_Start_Repair/06_Id_Iq_PI_and_Voltage_Circle/02_Voltage_Circle ==
  In1 : Inport
  Negative_Q_limit : Gain  Gain=-1
  Nonnegative_margin : Saturate  UpperLimit=inf  LowerLimit=0
  Q_voltage_limit : Math  Operator=sqrt
  Remaining_voltage : Sum  Inputs=+-
  Vd_squared : Math  Operator=square
  Voltage_circle_squared : Constant  Value=min(max(q.Vbus/12,0),0.95)^2
  Out1 : Outport
  Out2 : Outport  Port=2
  wires:
  In1/1 -> Vd_squared/1
  Voltage_circle_squared/1 -> Remaining_voltage/1
  Remaining_voltage/1 -> Nonnegative_margin/1
  Vd_squared/1 -> Remaining_voltage/2
  Negative_Q_limit/1 -> Out2/1
  Nonnegative_margin/1 -> Q_voltage_limit/1
  Q_voltage_limit/1 -> Out1/1, Negative_Q_limit/1

== system G474_Mode2_Direct_Start_Repair/06_Id_Iq_PI_and_Voltage_Circle/03_Iq_PI_and_Filter ==
  Ref : Inport
  Umax : Inport  Port=2
  Fbk : Inport  Port=3
  Umin : Inport  Port=4
  Iq_OutF : Sum
  Iq_OutF_new_01 : Gain  Gain=0.1
  Iq_OutF_old_09 : Gain  Gain=0.9
  Iq_OutF_previous : UnitDelay  SampleTime=p.Ts  HasFrameUpgradeWarning=on
  Iq_PI : Subsystem  mask{Kp=q.current_kp, Ki=q.current_ki, Ts=p.Ts}
      mask prompts: Kp "Kp (source coefficient)"; Ki "Ki (per call, already discrete)"; Ts "Execution period (s)"
      settings: OpenFcn=open_system(gcb,'force')
      mask Display: port_label('input',1,'Ref');port_label('input',2,'Fbk');port_label('input',3,'Umax');port_label('input',4,'Umin');port_label('output',1,'Out');port_label('output',2,'ui');port_label('output',3,'v1');port_label('output',4,'up');
  Out1 : Outport
  wires:
  Ref/1 -> Iq_PI/1(Ref)
  Fbk/1 -> Iq_PI/2(Fbk)
  Iq_OutF_new_01/1 -> Iq_OutF/2
  Umax/1 -> Iq_PI/3(Umax)
  Umin/1 -> Iq_PI/4(Umin)
  Iq_PI/1(Out) -> Iq_OutF_new_01/1
  Iq_OutF_previous/1 -> Iq_OutF_old_09/1
  Iq_OutF_old_09/1 -> Iq_OutF/1
  Iq_OutF/1 -> Iq_OutF_previous/1, Out1/1
